simulink model "six_pulse_dstack_based_rectifier"  (R2026a)
settings: Solver=ode23tb  StopTime=simlength  FixedStep=Ts  MaxStep=Tc  EnableMultiTasking=on
values from neighbouring files (symbols this model uses):
  Csnubber = 0.1e-6    (= 1e-07)    [init_model.m]
  LFu_dc = 1.2e-3    (= 0.0012)    [init_model.m]
  Rgrading = 2.4e6    (= 2400000)    [init_model.m]
  RLFu_dc = 2e-4    (= 0.0002)    [init_model.m]
  Rsnubber = 1000    [init_model.m]
  Tc = Tcontrol_rect/4000    (= 5e-08)    [init_model.m]
  Tcontrol_rect = tPWM_RECT    (= 0.0002)    [init_model.m]
  Vnom_ac_adc = 400/sqrt(3)*sqrt(2)    [init_model.m]
  w_grid = f_grid*2*pi    (= 314.159265359)    [init_model.m]
undefined symbols (not defined in the file or in its folder): magnitude, rms
libraries: fl_lib x179, nesl_utility x129, diode_rr_lib x36, ee_lib x2
(part 2 of 5)

== system six_pulse_dstack_based_rectifier/six_pulse rectifier/BR2/ssc_diode_rr_bridge/D1/D12 ==
  D12 : Subsystem
      settings: PortSchema="{\"entries\":[{\"content\":{\"sides\":[{\"content\":{},\"type\":\"ConnectorPlacement.EquallySpacedRectSide\",\"uuid\":\"7269b907-ab9b-4481-ac18-a8dd984c3818\"},{\"content\":{\"side\":\"RIGHT\"},\"type\":\"ConnectorPlacement.EquallySpacedRectSide\",\"uuid\":\"8dceca02-62a3-4342-b624-c7d4418298d0\"},{\"content\":{\"connectorIds\":[\"LConn1\"],\"side\":\"TOP\"},\"type\":\"ConnectorPlacement.EquallySpacedRectSide\",\"uuid\":\"a3401fa4-31f5-4c91-8a09-9f2730c54d6f\"},{\"content\":{\"connectorIds\":[\"RConn1\"],\"side\":\"BOTTOM\"},\"type\":\"ConnectorPlacement.EquallySpacedRectSide\",\"uuid\":\"ec3e6ca2-4822-4b63-8ee1-1049d14efe1d\"}]},\"type\":\"ConnectorPlacement.EquallySpacedConnector\",\"uuid\":\"06f44f8b-bef4-44e1-af36-23832e4d595a\"}],\"packageUris\":[\"http://schema.mathworks.com/mf0/Connector/R2020b\"],\"version\":\"1.0\"}"
  K : PMIOPort  Side=Right
  A : PMIOPort  Port=2  Side=Left
  connections:
  A/RConn1 -- D12/RConn1
  D12/LConn1 -- K/RConn1

== system six_pulse_dstack_based_rectifier/six_pulse rectifier/BR2/ssc_diode_rr_bridge/D1/D13 ==
  D13 : Subsystem
      settings: PortSchema="{\"entries\":[{\"content\":{\"sides\":[{\"content\":{},\"type\":\"ConnectorPlacement.EquallySpacedRectSide\",\"uuid\":\"7269b907-ab9b-4481-ac18-a8dd984c3818\"},{\"content\":{\"side\":\"RIGHT\"},\"type\":\"ConnectorPlacement.EquallySpacedRectSide\",\"uuid\":\"8dceca02-62a3-4342-b624-c7d4418298d0\"},{\"content\":{\"connectorIds\":[\"LConn1\"],\"side\":\"TOP\"},\"type\":\"ConnectorPlacement.EquallySpacedRectSide\",\"uuid\":\"a3401fa4-31f5-4c91-8a09-9f2730c54d6f\"},{\"content\":{\"connectorIds\":[\"RConn1\"],\"side\":\"BOTTOM\"},\"type\":\"ConnectorPlacement.EquallySpacedRectSide\",\"uuid\":\"ec3e6ca2-4822-4b63-8ee1-1049d14efe1d\"}]},\"type\":\"ConnectorPlacement.EquallySpacedConnector\",\"uuid\":\"06f44f8b-bef4-44e1-af36-23832e4d595a\"}],\"packageUris\":[\"http://schema.mathworks.com/mf0/Connector/R2020b\"],\"version\":\"1.0\"}"
  K : PMIOPort  Side=Right
  A : PMIOPort  Port=2  Side=Left
  connections:
  D13/LConn1 -- K/RConn1
  A/RConn1 -- D13/RConn1

== system six_pulse_dstack_based_rectifier/six_pulse rectifier/BR2/ssc_diode_rr_bridge/D1/D14 ==
  D14 : Subsystem
      settings: PortSchema="{\"entries\":[{\"content\":{\"sides\":[{\"content\":{},\"type\":\"ConnectorPlacement.EquallySpacedRectSide\",\"uuid\":\"7269b907-ab9b-4481-ac18-a8dd984c3818\"},{\"content\":{\"side\":\"RIGHT\"},\"type\":\"ConnectorPlacement.EquallySpacedRectSide\",\"uuid\":\"8dceca02-62a3-4342-b624-c7d4418298d0\"},{\"content\":{\"connectorIds\":[\"LConn1\"],\"side\":\"TOP\"},\"type\":\"ConnectorPlacement.EquallySpacedRectSide\",\"uuid\":\"a3401fa4-31f5-4c91-8a09-9f2730c54d6f\"},{\"content\":{\"connectorIds\":[\"RConn1\"],\"side\":\"BOTTOM\"},\"type\":\"ConnectorPlacement.EquallySpacedRectSide\",\"uuid\":\"ec3e6ca2-4822-4b63-8ee1-1049d14efe1d\"}]},\"type\":\"ConnectorPlacement.EquallySpacedConnector\",\"uuid\":\"06f44f8b-bef4-44e1-af36-23832e4d595a\"}],\"packageUris\":[\"http://schema.mathworks.com/mf0/Connector/R2020b\"],\"version\":\"1.0\"}"
  K : PMIOPort  Side=Right
  A : PMIOPort  Port=2  Side=Left
  connections:
  A/RConn1 -- D14/RConn1
  D14/LConn1 -- K/RConn1

== system six_pulse_dstack_based_rectifier/six_pulse rectifier/BR2/ssc_diode_rr_bridge/D1/D15 ==
  D15 : Subsystem
      settings: PortSchema="{\"entries\":[{\"content\":{\"sides\":[{\"content\":{},\"type\":\"ConnectorPlacement.EquallySpacedRectSide\",\"uuid\":\"7269b907-ab9b-4481-ac18-a8dd984c3818\"},{\"content\":{\"side\":\"RIGHT\"},\"type\":\"ConnectorPlacement.EquallySpacedRectSide\",\"uuid\":\"8dceca02-62a3-4342-b624-c7d4418298d0\"},{\"content\":{\"connectorIds\":[\"LConn1\"],\"side\":\"TOP\"},\"type\":\"ConnectorPlacement.EquallySpacedRectSide\",\"uuid\":\"a3401fa4-31f5-4c91-8a09-9f2730c54d6f\"},{\"content\":{\"connectorIds\":[\"RConn1\"],\"side\":\"BOTTOM\"},\"type\":\"ConnectorPlacement.EquallySpacedRectSide\",\"uuid\":\"ec3e6ca2-4822-4b63-8ee1-1049d14efe1d\"}]},\"type\":\"ConnectorPlacement.EquallySpacedConnector\",\"uuid\":\"06f44f8b-bef4-44e1-af36-23832e4d595a\"}],\"packageUris\":[\"http://schema.mathworks.com/mf0/Connector/R2020b\"],\"version\":\"1.0\"}"
  K : PMIOPort  Side=Right
  A : PMIOPort  Port=2  Side=Left
  connections:
  D15/LConn1 -- K/RConn1
  A/RConn1 -- D15/RConn1

== system six_pulse_dstack_based_rectifier/six_pulse rectifier/BR2/ssc_diode_rr_bridge/D1/D16 ==
  D16 : Subsystem
      settings: PortSchema="{\"entries\":[{\"content\":{\"sides\":[{\"content\":{},\"type\":\"ConnectorPlacement.EquallySpacedRectSide\",\"uuid\":\"7269b907-ab9b-4481-ac18-a8dd984c3818\"},{\"content\":{\"side\":\"RIGHT\"},\"type\":\"ConnectorPlacement.EquallySpacedRectSide\",\"uuid\":\"8dceca02-62a3-4342-b624-c7d4418298d0\"},{\"content\":{\"connectorIds\":[\"LConn1\"],\"side\":\"TOP\"},\"type\":\"ConnectorPlacement.EquallySpacedRectSide\",\"uuid\":\"a3401fa4-31f5-4c91-8a09-9f2730c54d6f\"},{\"content\":{\"connectorIds\":[\"RConn1\"],\"side\":\"BOTTOM\"},\"type\":\"ConnectorPlacement.EquallySpacedRectSide\",\"uuid\":\"ec3e6ca2-4822-4b63-8ee1-1049d14efe1d\"}]},\"type\":\"ConnectorPlacement.EquallySpacedConnector\",\"uuid\":\"06f44f8b-bef4-44e1-af36-23832e4d595a\"}],\"packageUris\":[\"http://schema.mathworks.com/mf0/Connector/R2020b\"],\"version\":\"1.0\"}"
  K : PMIOPort  Side=Right
  A : PMIOPort  Port=2  Side=Left
  connections:
  A/RConn1 -- D16/RConn1
  D16/LConn1 -- K/RConn1

== system six_pulse_dstack_based_rectifier/six_pulse rectifier/BR2/ssc_diode_rr_bridge/D1/Rgrading ==
  Current Sensor : fl_lib/Electrical/Electrical Sensors/Current Sensor
  PS-Simulink Converter : nesl_utility/PS-Simulink Converter  PhysicalDomain=network_engine_domain  SubClassName=ps_output  LeftPortType=input  RightPortType=output  PseudoPeriodic=off  Frequencies=[]  VectorFormat=inherit  Unit=inherit  AffineConversion=off
  PS-Simulink Converter1 : nesl_utility/PS-Simulink Converter  PhysicalDomain=network_engine_domain  SubClassName=ps_output  LeftPortType=input  RightPortType=output  PseudoPeriodic=off  Frequencies=[]  VectorFormat=inherit  Unit=inherit  AffineConversion=off
  R11 : fl_lib/Electrical/Electrical Elements/Resistor  R=Rgrading_m Ohm  i_specify=off  i_priority=None  i=0 A  i_nominal_specify=off  i_nominal_value=1  i_nominal_unit=A  v_specify=off  v_priority=None  v=0 V  v_nominal_specify=off  v_nominal_value=1  v_nominal_unit=V
  Voltage Sensor : fl_lib/Electrical/Electrical Sensors/Voltage Sensor
  K : PMIOPort  Side=Right
  A : PMIOPort  Port=2  Side=Left
  tag scope: Rg11_I=scoped, Rg11_U=scoped
  wires:
  PS-Simulink Converter/1 -> [Rg11_U]
  PS-Simulink Converter1/1 -> [Rg11_I]
  connections:
  Voltage Sensor/LConn1 -- Current Sensor/LConn1 -- A/RConn1
  R11/RConn1 -- Voltage Sensor/RConn2 -- K/RConn1
  PS-Simulink Converter/LConn1 -- Voltage Sensor/RConn1
  Current Sensor/RConn2 -- R11/LConn1
  Current Sensor/RConn1 -- PS-Simulink Converter1/LConn1

== system six_pulse_dstack_based_rectifier/six_pulse rectifier/BR2/ssc_diode_rr_bridge/D2/D11 ==
  D11 : Subsystem
      settings: PortSchema="{\"entries\":[{\"content\":{\"sides\":[{\"content\":{},\"type\":\"ConnectorPlacement.EquallySpacedRectSide\",\"uuid\":\"7269b907-ab9b-4481-ac18-a8dd984c3818\"},{\"content\":{\"side\":\"RIGHT\"},\"type\":\"ConnectorPlacement.EquallySpacedRectSide\",\"uuid\":\"8dceca02-62a3-4342-b624-c7d4418298d0\"},{\"content\":{\"connectorIds\":[\"LConn1\"],\"side\":\"TOP\"},\"type\":\"ConnectorPlacement.EquallySpacedRectSide\",\"uuid\":\"a3401fa4-31f5-4c91-8a09-9f2730c54d6f\"},{\"content\":{\"connectorIds\":[\"RConn1\"],\"side\":\"BOTTOM\"},\"type\":\"ConnectorPlacement.EquallySpacedRectSide\",\"uuid\":\"ec3e6ca2-4822-4b63-8ee1-1049d14efe1d\"}]},\"type\":\"ConnectorPlacement.EquallySpacedConnector\",\"uuid\":\"06f44f8b-bef4-44e1-af36-23832e4d595a\"}],\"packageUris\":[\"http://schema.mathworks.com/mf0/Connector/R2020b\"],\"version\":\"1.0\"}"
  K : PMIOPort  Side=Right
  A : PMIOPort  Port=2  Side=Left
  connections:
  A/RConn1 -- D11/RConn1
  D11/LConn1 -- K/RConn1

== system six_pulse_dstack_based_rectifier/six_pulse rectifier/BR2/ssc_diode_rr_bridge/D2/D12 ==
  D12 : Subsystem
      settings: PortSchema="{\"entries\":[{\"content\":{\"sides\":[{\"content\":{},\"type\":\"ConnectorPlacement.EquallySpacedRectSide\",\"uuid\":\"7269b907-ab9b-4481-ac18-a8dd984c3818\"},{\"content\":{\"side\":\"RIGHT\"},\"type\":\"ConnectorPlacement.EquallySpacedRectSide\",\"uuid\":\"8dceca02-62a3-4342-b624-c7d4418298d0\"},{\"content\":{\"connectorIds\":[\"LConn1\"],\"side\":\"TOP\"},\"type\":\"ConnectorPlacement.EquallySpacedRectSide\",\"uuid\":\"a3401fa4-31f5-4c91-8a09-9f2730c54d6f\"},{\"content\":{\"connectorIds\":[\"RConn1\"],\"side\":\"BOTTOM\"},\"type\":\"ConnectorPlacement.EquallySpacedRectSide\",\"uuid\":\"ec3e6ca2-4822-4b63-8ee1-1049d14efe1d\"}]},\"type\":\"ConnectorPlacement.EquallySpacedConnector\",\"uuid\":\"06f44f8b-bef4-44e1-af36-23832e4d595a\"}],\"packageUris\":[\"http://schema.mathworks.com/mf0/Connector/R2020b\"],\"version\":\"1.0\"}"
  K : PMIOPort  Side=Right
  A : PMIOPort  Port=2  Side=Left
  connections:
  D12/LConn1 -- K/RConn1
  A/RConn1 -- D12/RConn1

== system six_pulse_dstack_based_rectifier/six_pulse rectifier/BR2/ssc_diode_rr_bridge/D2/D13 ==
  D13 : Subsystem
      settings: PortSchema="{\"entries\":[{\"content\":{\"sides\":[{\"content\":{},\"type\":\"ConnectorPlacement.EquallySpacedRectSide\",\"uuid\":\"7269b907-ab9b-4481-ac18-a8dd984c3818\"},{\"content\":{\"side\":\"RIGHT\"},\"type\":\"ConnectorPlacement.EquallySpacedRectSide\",\"uuid\":\"8dceca02-62a3-4342-b624-c7d4418298d0\"},{\"content\":{\"connectorIds\":[\"LConn1\"],\"side\":\"TOP\"},\"type\":\"ConnectorPlacement.EquallySpacedRectSide\",\"uuid\":\"a3401fa4-31f5-4c91-8a09-9f2730c54d6f\"},{\"content\":{\"connectorIds\":[\"RConn1\"],\"side\":\"BOTTOM\"},\"type\":\"ConnectorPlacement.EquallySpacedRectSide\",\"uuid\":\"ec3e6ca2-4822-4b63-8ee1-1049d14efe1d\"}]},\"type\":\"ConnectorPlacement.EquallySpacedConnector\",\"uuid\":\"06f44f8b-bef4-44e1-af36-23832e4d595a\"}],\"packageUris\":[\"http://schema.mathworks.com/mf0/Connector/R2020b\"],\"version\":\"1.0\"}"
  K : PMIOPort  Side=Right
  A : PMIOPort  Port=2  Side=Left
  connections:
  A/RConn1 -- D13/RConn1
  D13/LConn1 -- K/RConn1

== system six_pulse_dstack_based_rectifier/six_pulse rectifier/BR2/ssc_diode_rr_bridge/D2/D14 ==
  D14 : Subsystem
      settings: PortSchema="{\"entries\":[{\"content\":{\"sides\":[{\"content\":{},\"type\":\"ConnectorPlacement.EquallySpacedRectSide\",\"uuid\":\"7269b907-ab9b-4481-ac18-a8dd984c3818\"},{\"content\":{\"side\":\"RIGHT\"},\"type\":\"ConnectorPlacement.EquallySpacedRectSide\",\"uuid\":\"8dceca02-62a3-4342-b624-c7d4418298d0\"},{\"content\":{\"connectorIds\":[\"LConn1\"],\"side\":\"TOP\"},\"type\":\"ConnectorPlacement.EquallySpacedRectSide\",\"uuid\":\"a3401fa4-31f5-4c91-8a09-9f2730c54d6f\"},{\"content\":{\"connectorIds\":[\"RConn1\"],\"side\":\"BOTTOM\"},\"type\":\"ConnectorPlacement.EquallySpacedRectSide\",\"uuid\":\"ec3e6ca2-4822-4b63-8ee1-1049d14efe1d\"}]},\"type\":\"ConnectorPlacement.EquallySpacedConnector\",\"uuid\":\"06f44f8b-bef4-44e1-af36-23832e4d595a\"}],\"packageUris\":[\"http://schema.mathworks.com/mf0/Connector/R2020b\"],\"version\":\"1.0\"}"
  K : PMIOPort  Side=Right
  A : PMIOPort  Port=2  Side=Left
  connections:
  D14/LConn1 -- K/RConn1
  A/RConn1 -- D14/RConn1

== system six_pulse_dstack_based_rectifier/six_pulse rectifier/BR2/ssc_diode_rr_bridge/D2/D15 ==
  D15 : Subsystem
      settings: PortSchema="{\"entries\":[{\"content\":{\"sides\":[{\"content\":{},\"type\":\"ConnectorPlacement.EquallySpacedRectSide\",\"uuid\":\"7269b907-ab9b-4481-ac18-a8dd984c3818\"},{\"content\":{\"side\":\"RIGHT\"},\"type\":\"ConnectorPlacement.EquallySpacedRectSide\",\"uuid\":\"8dceca02-62a3-4342-b624-c7d4418298d0\"},{\"content\":{\"connectorIds\":[\"LConn1\"],\"side\":\"TOP\"},\"type\":\"ConnectorPlacement.EquallySpacedRectSide\",\"uuid\":\"a3401fa4-31f5-4c91-8a09-9f2730c54d6f\"},{\"content\":{\"connectorIds\":[\"RConn1\"],\"side\":\"BOTTOM\"},\"type\":\"ConnectorPlacement.EquallySpacedRectSide\",\"uuid\":\"ec3e6ca2-4822-4b63-8ee1-1049d14efe1d\"}]},\"type\":\"ConnectorPlacement.EquallySpacedConnector\",\"uuid\":\"06f44f8b-bef4-44e1-af36-23832e4d595a\"}],\"packageUris\":[\"http://schema.mathworks.com/mf0/Connector/R2020b\"],\"version\":\"1.0\"}"
  K : PMIOPort  Side=Right
  A : PMIOPort  Port=2  Side=Left
  connections:
  A/RConn1 -- D15/RConn1
  D15/LConn1 -- K/RConn1

== system six_pulse_dstack_based_rectifier/six_pulse rectifier/BR2/ssc_diode_rr_bridge/D2/D16 ==
  D16 : Subsystem
      settings: PortSchema="{\"entries\":[{\"content\":{\"sides\":[{\"content\":{},\"type\":\"ConnectorPlacement.EquallySpacedRectSide\",\"uuid\":\"7269b907-ab9b-4481-ac18-a8dd984c3818\"},{\"content\":{\"side\":\"RIGHT\"},\"type\":\"ConnectorPlacement.EquallySpacedRectSide\",\"uuid\":\"8dceca02-62a3-4342-b624-c7d4418298d0\"},{\"content\":{\"connectorIds\":[\"LConn1\"],\"side\":\"TOP\"},\"type\":\"ConnectorPlacement.EquallySpacedRectSide\",\"uuid\":\"a3401fa4-31f5-4c91-8a09-9f2730c54d6f\"},{\"content\":{\"connectorIds\":[\"RConn1\"],\"side\":\"BOTTOM\"},\"type\":\"ConnectorPlacement.EquallySpacedRectSide\",\"uuid\":\"ec3e6ca2-4822-4b63-8ee1-1049d14efe1d\"}]},\"type\":\"ConnectorPlacement.EquallySpacedConnector\",\"uuid\":\"06f44f8b-bef4-44e1-af36-23832e4d595a\"}],\"packageUris\":[\"http://schema.mathworks.com/mf0/Connector/R2020b\"],\"version\":\"1.0\"}"
  K : PMIOPort  Side=Right
  A : PMIOPort  Port=2  Side=Left
  connections:
  D16/LConn1 -- K/RConn1
  A/RConn1 -- D16/RConn1

== system six_pulse_dstack_based_rectifier/six_pulse rectifier/BR2/ssc_diode_rr_bridge/D3/D11 ==
  D11 : Subsystem
      settings: PortSchema="{\"entries\":[{\"content\":{\"sides\":[{\"content\":{},\"type\":\"ConnectorPlacement.EquallySpacedRectSide\",\"uuid\":\"7269b907-ab9b-4481-ac18-a8dd984c3818\"},{\"content\":{\"side\":\"RIGHT\"},\"type\":\"ConnectorPlacement.EquallySpacedRectSide\",\"uuid\":\"8dceca02-62a3-4342-b624-c7d4418298d0\"},{\"content\":{\"connectorIds\":[\"LConn1\"],\"side\":\"TOP\"},\"type\":\"ConnectorPlacement.EquallySpacedRectSide\",\"uuid\":\"a3401fa4-31f5-4c91-8a09-9f2730c54d6f\"},{\"content\":{\"connectorIds\":[\"RConn1\"],\"side\":\"BOTTOM\"},\"type\":\"ConnectorPlacement.EquallySpacedRectSide\",\"uuid\":\"ec3e6ca2-4822-4b63-8ee1-1049d14efe1d\"}]},\"type\":\"ConnectorPlacement.EquallySpacedConnector\",\"uuid\":\"06f44f8b-bef4-44e1-af36-23832e4d595a\"}],\"packageUris\":[\"http://schema.mathworks.com/mf0/Connector/R2020b\"],\"version\":\"1.0\"}"
  K : PMIOPort  Side=Right
  A : PMIOPort  Port=2  Side=Left
  connections:
  A/RConn1 -- D11/RConn1
  D11/LConn1 -- K/RConn1

== system six_pulse_dstack_based_rectifier/six_pulse rectifier/BR2/ssc_diode_rr_bridge/D3/D12 ==
  D12 : Subsystem
      settings: PortSchema="{\"entries\":[{\"content\":{\"sides\":[{\"content\":{},\"type\":\"ConnectorPlacement.EquallySpacedRectSide\",\"uuid\":\"7269b907-ab9b-4481-ac18-a8dd984c3818\"},{\"content\":{\"side\":\"RIGHT\"},\"type\":\"ConnectorPlacement.EquallySpacedRectSide\",\"uuid\":\"8dceca02-62a3-4342-b624-c7d4418298d0\"},{\"content\":{\"connectorIds\":[\"LConn1\"],\"side\":\"TOP\"},\"type\":\"ConnectorPlacement.EquallySpacedRectSide\",\"uuid\":\"a3401fa4-31f5-4c91-8a09-9f2730c54d6f\"},{\"content\":{\"connectorIds\":[\"RConn1\"],\"side\":\"BOTTOM\"},\"type\":\"ConnectorPlacement.EquallySpacedRectSide\",\"uuid\":\"ec3e6ca2-4822-4b63-8ee1-1049d14efe1d\"}]},\"type\":\"ConnectorPlacement.EquallySpacedConnector\",\"uuid\":\"06f44f8b-bef4-44e1-af36-23832e4d595a\"}],\"packageUris\":[\"http://schema.mathworks.com/mf0/Connector/R2020b\"],\"version\":\"1.0\"}"
  K : PMIOPort  Side=Right
  A : PMIOPort  Port=2  Side=Left
  connections:
  D12/LConn1 -- K/RConn1
  A/RConn1 -- D12/RConn1

== system six_pulse_dstack_based_rectifier/six_pulse rectifier/BR2/ssc_diode_rr_bridge/D3/D13 ==
  D13 : Subsystem
      settings: PortSchema="{\"entries\":[{\"content\":{\"sides\":[{\"content\":{},\"type\":\"ConnectorPlacement.EquallySpacedRectSide\",\"uuid\":\"7269b907-ab9b-4481-ac18-a8dd984c3818\"},{\"content\":{\"side\":\"RIGHT\"},\"type\":\"ConnectorPlacement.EquallySpacedRectSide\",\"uuid\":\"8dceca02-62a3-4342-b624-c7d4418298d0\"},{\"content\":{\"connectorIds\":[\"LConn1\"],\"side\":\"TOP\"},\"type\":\"ConnectorPlacement.EquallySpacedRectSide\",\"uuid\":\"a3401fa4-31f5-4c91-8a09-9f2730c54d6f\"},{\"content\":{\"connectorIds\":[\"RConn1\"],\"side\":\"BOTTOM\"},\"type\":\"ConnectorPlacement.EquallySpacedRectSide\",\"uuid\":\"ec3e6ca2-4822-4b63-8ee1-1049d14efe1d\"}]},\"type\":\"ConnectorPlacement.EquallySpacedConnector\",\"uuid\":\"06f44f8b-bef4-44e1-af36-23832e4d595a\"}],\"packageUris\":[\"http://schema.mathworks.com/mf0/Connector/R2020b\"],\"version\":\"1.0\"}"
  K : PMIOPort  Side=Right
  A : PMIOPort  Port=2  Side=Left
  connections:
  A/RConn1 -- D13/RConn1
  D13/LConn1 -- K/RConn1

== system six_pulse_dstack_based_rectifier/six_pulse rectifier/BR2/ssc_diode_rr_bridge/D3/D14 ==
  D14 : Subsystem
      settings: PortSchema="{\"entries\":[{\"content\":{\"sides\":[{\"content\":{},\"type\":\"ConnectorPlacement.EquallySpacedRectSide\",\"uuid\":\"7269b907-ab9b-4481-ac18-a8dd984c3818\"},{\"content\":{\"side\":\"RIGHT\"},\"type\":\"ConnectorPlacement.EquallySpacedRectSide\",\"uuid\":\"8dceca02-62a3-4342-b624-c7d4418298d0\"},{\"content\":{\"connectorIds\":[\"LConn1\"],\"side\":\"TOP\"},\"type\":\"ConnectorPlacement.EquallySpacedRectSide\",\"uuid\":\"a3401fa4-31f5-4c91-8a09-9f2730c54d6f\"},{\"content\":{\"connectorIds\":[\"RConn1\"],\"side\":\"BOTTOM\"},\"type\":\"ConnectorPlacement.EquallySpacedRectSide\",\"uuid\":\"ec3e6ca2-4822-4b63-8ee1-1049d14efe1d\"}]},\"type\":\"ConnectorPlacement.EquallySpacedConnector\",\"uuid\":\"06f44f8b-bef4-44e1-af36-23832e4d595a\"}],\"packageUris\":[\"http://schema.mathworks.com/mf0/Connector/R2020b\"],\"version\":\"1.0\"}"
  K : PMIOPort  Side=Right
  A : PMIOPort  Port=2  Side=Left
  connections:
  D14/LConn1 -- K/RConn1
  A/RConn1 -- D14/RConn1

== system six_pulse_dstack_based_rectifier/six_pulse rectifier/BR2/ssc_diode_rr_bridge/D3/D15 ==
  D15 : Subsystem
      settings: PortSchema="{\"entries\":[{\"content\":{\"sides\":[{\"content\":{},\"type\":\"ConnectorPlacement.EquallySpacedRectSide\",\"uuid\":\"7269b907-ab9b-4481-ac18-a8dd984c3818\"},{\"content\":{\"side\":\"RIGHT\"},\"type\":\"ConnectorPlacement.EquallySpacedRectSide\",\"uuid\":\"8dceca02-62a3-4342-b624-c7d4418298d0\"},{\"content\":{\"connectorIds\":[\"LConn1\"],\"side\":\"TOP\"},\"type\":\"ConnectorPlacement.EquallySpacedRectSide\",\"uuid\":\"a3401fa4-31f5-4c91-8a09-9f2730c54d6f\"},{\"content\":{\"connectorIds\":[\"RConn1\"],\"side\":\"BOTTOM\"},\"type\":\"ConnectorPlacement.EquallySpacedRectSide\",\"uuid\":\"ec3e6ca2-4822-4b63-8ee1-1049d14efe1d\"}]},\"type\":\"ConnectorPlacement.EquallySpacedConnector\",\"uuid\":\"06f44f8b-bef4-44e1-af36-23832e4d595a\"}],\"packageUris\":[\"http://schema.mathworks.com/mf0/Connector/R2020b\"],\"version\":\"1.0\"}"
  K : PMIOPort  Side=Right
  A : PMIOPort  Port=2  Side=Left
  connections:
  A/RConn1 -- D15/RConn1
  D15/LConn1 -- K/RConn1

== system six_pulse_dstack_based_rectifier/six_pulse rectifier/BR2/ssc_diode_rr_bridge/D3/D16 ==
  D16 : Subsystem
      settings: PortSchema="{\"entries\":[{\"content\":{\"sides\":[{\"content\":{},\"type\":\"ConnectorPlacement.EquallySpacedRectSide\",\"uuid\":\"7269b907-ab9b-4481-ac18-a8dd984c3818\"},{\"content\":{\"side\":\"RIGHT\"},\"type\":\"ConnectorPlacement.EquallySpacedRectSide\",\"uuid\":\"8dceca02-62a3-4342-b624-c7d4418298d0\"},{\"content\":{\"connectorIds\":[\"LConn1\"],\"side\":\"TOP\"},\"type\":\"ConnectorPlacement.EquallySpacedRectSide\",\"uuid\":\"a3401fa4-31f5-4c91-8a09-9f2730c54d6f\"},{\"content\":{\"connectorIds\":[\"RConn1\"],\"side\":\"BOTTOM\"},\"type\":\"ConnectorPlacement.EquallySpacedRectSide\",\"uuid\":\"ec3e6ca2-4822-4b63-8ee1-1049d14efe1d\"}]},\"type\":\"ConnectorPlacement.EquallySpacedConnector\",\"uuid\":\"06f44f8b-bef4-44e1-af36-23832e4d595a\"}],\"packageUris\":[\"http://schema.mathworks.com/mf0/Connector/R2020b\"],\"version\":\"1.0\"}"
  K : PMIOPort  Side=Right
  A : PMIOPort  Port=2  Side=Left
  connections:
  D16/LConn1 -- K/RConn1
  A/RConn1 -- D16/RConn1

== system six_pulse_dstack_based_rectifier/six_pulse rectifier/BR2/ssc_diode_rr_bridge/D4/D11 ==
  D11 : Subsystem
      settings: PortSchema="{\"entries\":[{\"content\":{\"sides\":[{\"content\":{},\"type\":\"ConnectorPlacement.EquallySpacedRectSide\",\"uuid\":\"7269b907-ab9b-4481-ac18-a8dd984c3818\"},{\"content\":{\"side\":\"RIGHT\"},\"type\":\"ConnectorPlacement.EquallySpacedRectSide\",\"uuid\":\"8dceca02-62a3-4342-b624-c7d4418298d0\"},{\"content\":{\"connectorIds\":[\"LConn1\"],\"side\":\"TOP\"},\"type\":\"ConnectorPlacement.EquallySpacedRectSide\",\"uuid\":\"a3401fa4-31f5-4c91-8a09-9f2730c54d6f\"},{\"content\":{\"connectorIds\":[\"RConn1\"],\"side\":\"BOTTOM\"},\"type\":\"ConnectorPlacement.EquallySpacedRectSide\",\"uuid\":\"ec3e6ca2-4822-4b63-8ee1-1049d14efe1d\"}]},\"type\":\"ConnectorPlacement.EquallySpacedConnector\",\"uuid\":\"06f44f8b-bef4-44e1-af36-23832e4d595a\"}],\"packageUris\":[\"http://schema.mathworks.com/mf0/Connector/R2020b\"],\"version\":\"1.0\"}"
  K : PMIOPort  Side=Right
  A : PMIOPort  Port=2  Side=Left
  connections:
  D11/LConn1 -- K/RConn1
  A/RConn1 -- D11/RConn1

== system six_pulse_dstack_based_rectifier/six_pulse rectifier/BR2/ssc_diode_rr_bridge/D4/D12 ==
  D12 : Subsystem
      settings: PortSchema="{\"entries\":[{\"content\":{\"sides\":[{\"content\":{},\"type\":\"ConnectorPlacement.EquallySpacedRectSide\",\"uuid\":\"7269b907-ab9b-4481-ac18-a8dd984c3818\"},{\"content\":{\"side\":\"RIGHT\"},\"type\":\"ConnectorPlacement.EquallySpacedRectSide\",\"uuid\":\"8dceca02-62a3-4342-b624-c7d4418298d0\"},{\"content\":{\"connectorIds\":[\"LConn1\"],\"side\":\"TOP\"},\"type\":\"ConnectorPlacement.EquallySpacedRectSide\",\"uuid\":\"a3401fa4-31f5-4c91-8a09-9f2730c54d6f\"},{\"content\":{\"connectorIds\":[\"RConn1\"],\"side\":\"BOTTOM\"},\"type\":\"ConnectorPlacement.EquallySpacedRectSide\",\"uuid\":\"ec3e6ca2-4822-4b63-8ee1-1049d14efe1d\"}]},\"type\":\"ConnectorPlacement.EquallySpacedConnector\",\"uuid\":\"06f44f8b-bef4-44e1-af36-23832e4d595a\"}],\"packageUris\":[\"http://schema.mathworks.com/mf0/Connector/R2020b\"],\"version\":\"1.0\"}"
  K : PMIOPort  Side=Right
  A : PMIOPort  Port=2  Side=Left
  connections:
  A/RConn1 -- D12/RConn1
  D12/LConn1 -- K/RConn1

== system six_pulse_dstack_based_rectifier/six_pulse rectifier/BR2/ssc_diode_rr_bridge/D4/D13 ==
  D13 : Subsystem
      settings: PortSchema="{\"entries\":[{\"content\":{\"sides\":[{\"content\":{},\"type\":\"ConnectorPlacement.EquallySpacedRectSide\",\"uuid\":\"7269b907-ab9b-4481-ac18-a8dd984c3818\"},{\"content\":{\"side\":\"RIGHT\"},\"type\":\"ConnectorPlacement.EquallySpacedRectSide\",\"uuid\":\"8dceca02-62a3-4342-b624-c7d4418298d0\"},{\"content\":{\"connectorIds\":[\"LConn1\"],\"side\":\"TOP\"},\"type\":\"ConnectorPlacement.EquallySpacedRectSide\",\"uuid\":\"a3401fa4-31f5-4c91-8a09-9f2730c54d6f\"},{\"content\":{\"connectorIds\":[\"RConn1\"],\"side\":\"BOTTOM\"},\"type\":\"ConnectorPlacement.EquallySpacedRectSide\",\"uuid\":\"ec3e6ca2-4822-4b63-8ee1-1049d14efe1d\"}]},\"type\":\"ConnectorPlacement.EquallySpacedConnector\",\"uuid\":\"06f44f8b-bef4-44e1-af36-23832e4d595a\"}],\"packageUris\":[\"http://schema.mathworks.com/mf0/Connector/R2020b\"],\"version\":\"1.0\"}"
  K : PMIOPort  Side=Right
  A : PMIOPort  Port=2  Side=Left
  connections:
  D13/LConn1 -- K/RConn1
  A/RConn1 -- D13/RConn1

== system six_pulse_dstack_based_rectifier/six_pulse rectifier/BR2/ssc_diode_rr_bridge/D4/D14 ==
  D14 : Subsystem
      settings: PortSchema="{\"entries\":[{\"content\":{\"sides\":[{\"content\":{},\"type\":\"ConnectorPlacement.EquallySpacedRectSide\",\"uuid\":\"7269b907-ab9b-4481-ac18-a8dd984c3818\"},{\"content\":{\"side\":\"RIGHT\"},\"type\":\"ConnectorPlacement.EquallySpacedRectSide\",\"uuid\":\"8dceca02-62a3-4342-b624-c7d4418298d0\"},{\"content\":{\"connectorIds\":[\"LConn1\"],\"side\":\"TOP\"},\"type\":\"ConnectorPlacement.EquallySpacedRectSide\",\"uuid\":\"a3401fa4-31f5-4c91-8a09-9f2730c54d6f\"},{\"content\":{\"connectorIds\":[\"RConn1\"],\"side\":\"BOTTOM\"},\"type\":\"ConnectorPlacement.EquallySpacedRectSide\",\"uuid\":\"ec3e6ca2-4822-4b63-8ee1-1049d14efe1d\"}]},\"type\":\"ConnectorPlacement.EquallySpacedConnector\",\"uuid\":\"06f44f8b-bef4-44e1-af36-23832e4d595a\"}],\"packageUris\":[\"http://schema.mathworks.com/mf0/Connector/R2020b\"],\"version\":\"1.0\"}"
  K : PMIOPort  Side=Right
  A : PMIOPort  Port=2  Side=Left
  connections:
  A/RConn1 -- D14/RConn1
  D14/LConn1 -- K/RConn1

== system six_pulse_dstack_based_rectifier/six_pulse rectifier/BR2/ssc_diode_rr_bridge/D4/D15 ==
  D15 : Subsystem
      settings: PortSchema="{\"entries\":[{\"content\":{\"sides\":[{\"content\":{},\"type\":\"ConnectorPlacement.EquallySpacedRectSide\",\"uuid\":\"7269b907-ab9b-4481-ac18-a8dd984c3818\"},{\"content\":{\"side\":\"RIGHT\"},\"type\":\"ConnectorPlacement.EquallySpacedRectSide\",\"uuid\":\"8dceca02-62a3-4342-b624-c7d4418298d0\"},{\"content\":{\"connectorIds\":[\"LConn1\"],\"side\":\"TOP\"},\"type\":\"ConnectorPlacement.EquallySpacedRectSide\",\"uuid\":\"a3401fa4-31f5-4c91-8a09-9f2730c54d6f\"},{\"content\":{\"connectorIds\":[\"RConn1\"],\"side\":\"BOTTOM\"},\"type\":\"ConnectorPlacement.EquallySpacedRectSide\",\"uuid\":\"ec3e6ca2-4822-4b63-8ee1-1049d14efe1d\"}]},\"type\":\"ConnectorPlacement.EquallySpacedConnector\",\"uuid\":\"06f44f8b-bef4-44e1-af36-23832e4d595a\"}],\"packageUris\":[\"http://schema.mathworks.com/mf0/Connector/R2020b\"],\"version\":\"1.0\"}"
  K : PMIOPort  Side=Right
  A : PMIOPort  Port=2  Side=Left
  connections:
  D15/LConn1 -- K/RConn1
  A/RConn1 -- D15/RConn1

== system six_pulse_dstack_based_rectifier/six_pulse rectifier/BR2/ssc_diode_rr_bridge/D4/D16 ==
  D16 : Subsystem
      settings: PortSchema="{\"entries\":[{\"content\":{\"sides\":[{\"content\":{},\"type\":\"ConnectorPlacement.EquallySpacedRectSide\",\"uuid\":\"7269b907-ab9b-4481-ac18-a8dd984c3818\"},{\"content\":{\"side\":\"RIGHT\"},\"type\":\"ConnectorPlacement.EquallySpacedRectSide\",\"uuid\":\"8dceca02-62a3-4342-b624-c7d4418298d0\"},{\"content\":{\"connectorIds\":[\"LConn1\"],\"side\":\"TOP\"},\"type\":\"ConnectorPlacement.EquallySpacedRectSide\",\"uuid\":\"a3401fa4-31f5-4c91-8a09-9f2730c54d6f\"},{\"content\":{\"connectorIds\":[\"RConn1\"],\"side\":\"BOTTOM\"},\"type\":\"ConnectorPlacement.EquallySpacedRectSide\",\"uuid\":\"ec3e6ca2-4822-4b63-8ee1-1049d14efe1d\"}]},\"type\":\"ConnectorPlacement.EquallySpacedConnector\",\"uuid\":\"06f44f8b-bef4-44e1-af36-23832e4d595a\"}],\"packageUris\":[\"http://schema.mathworks.com/mf0/Connector/R2020b\"],\"version\":\"1.0\"}"
  K : PMIOPort  Side=Right
  A : PMIOPort  Port=2  Side=Left
  connections:
  A/RConn1 -- D16/RConn1
  D16/LConn1 -- K/RConn1

== system six_pulse_dstack_based_rectifier/six_pulse rectifier/BR2/ssc_diode_rr_bridge/D5/D11 ==
  D11 : Subsystem
      settings: PortSchema="{\"entries\":[{\"content\":{\"sides\":[{\"content\":{},\"type\":\"ConnectorPlacement.EquallySpacedRectSide\",\"uuid\":\"7269b907-ab9b-4481-ac18-a8dd984c3818\"},{\"content\":{\"side\":\"RIGHT\"},\"type\":\"ConnectorPlacement.EquallySpacedRectSide\",\"uuid\":\"8dceca02-62a3-4342-b624-c7d4418298d0\"},{\"content\":{\"connectorIds\":[\"LConn1\"],\"side\":\"TOP\"},\"type\":\"ConnectorPlacement.EquallySpacedRectSide\",\"uuid\":\"a3401fa4-31f5-4c91-8a09-9f2730c54d6f\"},{\"content\":{\"connectorIds\":[\"RConn1\"],\"side\":\"BOTTOM\"},\"type\":\"ConnectorPlacement.EquallySpacedRectSide\",\"uuid\":\"ec3e6ca2-4822-4b63-8ee1-1049d14efe1d\"}]},\"type\":\"ConnectorPlacement.EquallySpacedConnector\",\"uuid\":\"06f44f8b-bef4-44e1-af36-23832e4d595a\"}],\"packageUris\":[\"http://schema.mathworks.com/mf0/Connector/R2020b\"],\"version\":\"1.0\"}"
  K : PMIOPort  Side=Right
  A : PMIOPort  Port=2  Side=Left
  connections:
  D11/LConn1 -- K/RConn1
  A/RConn1 -- D11/RConn1

== system six_pulse_dstack_based_rectifier/six_pulse rectifier/BR2/ssc_diode_rr_bridge/D5/D12 ==
  D12 : Subsystem
      settings: PortSchema="{\"entries\":[{\"content\":{\"sides\":[{\"content\":{},\"type\":\"ConnectorPlacement.EquallySpacedRectSide\",\"uuid\":\"7269b907-ab9b-4481-ac18-a8dd984c3818\"},{\"content\":{\"side\":\"RIGHT\"},\"type\":\"ConnectorPlacement.EquallySpacedRectSide\",\"uuid\":\"8dceca02-62a3-4342-b624-c7d4418298d0\"},{\"content\":{\"connectorIds\":[\"LConn1\"],\"side\":\"TOP\"},\"type\":\"ConnectorPlacement.EquallySpacedRectSide\",\"uuid\":\"a3401fa4-31f5-4c91-8a09-9f2730c54d6f\"},{\"content\":{\"connectorIds\":[\"RConn1\"],\"side\":\"BOTTOM\"},\"type\":\"ConnectorPlacement.EquallySpacedRectSide\",\"uuid\":\"ec3e6ca2-4822-4b63-8ee1-1049d14efe1d\"}]},\"type\":\"ConnectorPlacement.EquallySpacedConnector\",\"uuid\":\"06f44f8b-bef4-44e1-af36-23832e4d595a\"}],\"packageUris\":[\"http://schema.mathworks.com/mf0/Connector/R2020b\"],\"version\":\"1.0\"}"
  K : PMIOPort  Side=Right
  A : PMIOPort  Port=2  Side=Left
  connections:
  A/RConn1 -- D12/RConn1
  D12/LConn1 -- K/RConn1

== system six_pulse_dstack_based_rectifier/six_pulse rectifier/BR2/ssc_diode_rr_bridge/D5/D13 ==
  D13 : Subsystem
      settings: PortSchema="{\"entries\":[{\"content\":{\"sides\":[{\"content\":{},\"type\":\"ConnectorPlacement.EquallySpacedRectSide\",\"uuid\":\"7269b907-ab9b-4481-ac18-a8dd984c3818\"},{\"content\":{\"side\":\"RIGHT\"},\"type\":\"ConnectorPlacement.EquallySpacedRectSide\",\"uuid\":\"8dceca02-62a3-4342-b624-c7d4418298d0\"},{\"content\":{\"connectorIds\":[\"LConn1\"],\"side\":\"TOP\"},\"type\":\"ConnectorPlacement.EquallySpacedRectSide\",\"uuid\":\"a3401fa4-31f5-4c91-8a09-9f2730c54d6f\"},{\"content\":{\"connectorIds\":[\"RConn1\"],\"side\":\"BOTTOM\"},\"type\":\"ConnectorPlacement.EquallySpacedRectSide\",\"uuid\":\"ec3e6ca2-4822-4b63-8ee1-1049d14efe1d\"}]},\"type\":\"ConnectorPlacement.EquallySpacedConnector\",\"uuid\":\"06f44f8b-bef4-44e1-af36-23832e4d595a\"}],\"packageUris\":[\"http://schema.mathworks.com/mf0/Connector/R2020b\"],\"version\":\"1.0\"}"
  K : PMIOPort  Side=Right
  A : PMIOPort  Port=2  Side=Left
  connections:
  D13/LConn1 -- K/RConn1
  A/RConn1 -- D13/RConn1

== system six_pulse_dstack_based_rectifier/six_pulse rectifier/BR2/ssc_diode_rr_bridge/D5/D14 ==
  D14 : Subsystem
      settings: PortSchema="{\"entries\":[{\"content\":{\"sides\":[{\"content\":{},\"type\":\"ConnectorPlacement.EquallySpacedRectSide\",\"uuid\":\"7269b907-ab9b-4481-ac18-a8dd984c3818\"},{\"content\":{\"side\":\"RIGHT\"},\"type\":\"ConnectorPlacement.EquallySpacedRectSide\",\"uuid\":\"8dceca02-62a3-4342-b624-c7d4418298d0\"},{\"content\":{\"connectorIds\":[\"LConn1\"],\"side\":\"TOP\"},\"type\":\"ConnectorPlacement.EquallySpacedRectSide\",\"uuid\":\"a3401fa4-31f5-4c91-8a09-9f2730c54d6f\"},{\"content\":{\"connectorIds\":[\"RConn1\"],\"side\":\"BOTTOM\"},\"type\":\"ConnectorPlacement.EquallySpacedRectSide\",\"uuid\":\"ec3e6ca2-4822-4b63-8ee1-1049d14efe1d\"}]},\"type\":\"ConnectorPlacement.EquallySpacedConnector\",\"uuid\":\"06f44f8b-bef4-44e1-af36-23832e4d595a\"}],\"packageUris\":[\"http://schema.mathworks.com/mf0/Connector/R2020b\"],\"version\":\"1.0\"}"
  K : PMIOPort  Side=Right
  A : PMIOPort  Port=2  Side=Left
  connections:
  A/RConn1 -- D14/RConn1
  D14/LConn1 -- K/RConn1

== system six_pulse_dstack_based_rectifier/six_pulse rectifier/BR2/ssc_diode_rr_bridge/D5/D15 ==
  D15 : Subsystem
      settings: PortSchema="{\"entries\":[{\"content\":{\"sides\":[{\"content\":{},\"type\":\"ConnectorPlacement.EquallySpacedRectSide\",\"uuid\":\"7269b907-ab9b-4481-ac18-a8dd984c3818\"},{\"content\":{\"side\":\"RIGHT\"},\"type\":\"ConnectorPlacement.EquallySpacedRectSide\",\"uuid\":\"8dceca02-62a3-4342-b624-c7d4418298d0\"},{\"content\":{\"connectorIds\":[\"LConn1\"],\"side\":\"TOP\"},\"type\":\"ConnectorPlacement.EquallySpacedRectSide\",\"uuid\":\"a3401fa4-31f5-4c91-8a09-9f2730c54d6f\"},{\"content\":{\"connectorIds\":[\"RConn1\"],\"side\":\"BOTTOM\"},\"type\":\"ConnectorPlacement.EquallySpacedRectSide\",\"uuid\":\"ec3e6ca2-4822-4b63-8ee1-1049d14efe1d\"}]},\"type\":\"ConnectorPlacement.EquallySpacedConnector\",\"uuid\":\"06f44f8b-bef4-44e1-af36-23832e4d595a\"}],\"packageUris\":[\"http://schema.mathworks.com/mf0/Connector/R2020b\"],\"version\":\"1.0\"}"
  K : PMIOPort  Side=Right
  A : PMIOPort  Port=2  Side=Left
  connections:
  D15/LConn1 -- K/RConn1
  A/RConn1 -- D15/RConn1

== system six_pulse_dstack_based_rectifier/six_pulse rectifier/BR2/ssc_diode_rr_bridge/D5/D16 ==
  D16 : Subsystem
      settings: PortSchema="{\"entries\":[{\"content\":{\"sides\":[{\"content\":{},\"type\":\"ConnectorPlacement.EquallySpacedRectSide\",\"uuid\":\"7269b907-ab9b-4481-ac18-a8dd984c3818\"},{\"content\":{\"side\":\"RIGHT\"},\"type\":\"ConnectorPlacement.EquallySpacedRectSide\",\"uuid\":\"8dceca02-62a3-4342-b624-c7d4418298d0\"},{\"content\":{\"connectorIds\":[\"LConn1\"],\"side\":\"TOP\"},\"type\":\"ConnectorPlacement.EquallySpacedRectSide\",\"uuid\":\"a3401fa4-31f5-4c91-8a09-9f2730c54d6f\"},{\"content\":{\"connectorIds\":[\"RConn1\"],\"side\":\"BOTTOM\"},\"type\":\"ConnectorPlacement.EquallySpacedRectSide\",\"uuid\":\"ec3e6ca2-4822-4b63-8ee1-1049d14efe1d\"}]},\"type\":\"ConnectorPlacement.EquallySpacedConnector\",\"uuid\":\"06f44f8b-bef4-44e1-af36-23832e4d595a\"}],\"packageUris\":[\"http://schema.mathworks.com/mf0/Connector/R2020b\"],\"version\":\"1.0\"}"
  K : PMIOPort  Side=Right
  A : PMIOPort  Port=2  Side=Left
  connections:
  A/RConn1 -- D16/RConn1
  D16/LConn1 -- K/RConn1

== system six_pulse_dstack_based_rectifier/six_pulse rectifier/BR2/ssc_diode_rr_bridge/D6/D11 ==
  D11 : Subsystem
      settings: PortSchema="{\"entries\":[{\"content\":{\"sides\":[{\"content\":{},\"type\":\"ConnectorPlacement.EquallySpacedRectSide\",\"uuid\":\"7269b907-ab9b-4481-ac18-a8dd984c3818\"},{\"content\":{\"side\":\"RIGHT\"},\"type\":\"ConnectorPlacement.EquallySpacedRectSide\",\"uuid\":\"8dceca02-62a3-4342-b624-c7d4418298d0\"},{\"content\":{\"connectorIds\":[\"LConn1\"],\"side\":\"TOP\"},\"type\":\"ConnectorPlacement.EquallySpacedRectSide\",\"uuid\":\"a3401fa4-31f5-4c91-8a09-9f2730c54d6f\"},{\"content\":{\"connectorIds\":[\"RConn1\"],\"side\":\"BOTTOM\"},\"type\":\"ConnectorPlacement.EquallySpacedRectSide\",\"uuid\":\"ec3e6ca2-4822-4b63-8ee1-1049d14efe1d\"}]},\"type\":\"ConnectorPlacement.EquallySpacedConnector\",\"uuid\":\"06f44f8b-bef4-44e1-af36-23832e4d595a\"}],\"packageUris\":[\"http://schema.mathworks.com/mf0/Connector/R2020b\"],\"version\":\"1.0\"}"
  K : PMIOPort  Side=Right
  A : PMIOPort  Port=2  Side=Left
  connections:
  A/RConn1 -- D11/RConn1
  D11/LConn1 -- K/RConn1

== system six_pulse_dstack_based_rectifier/six_pulse rectifier/BR2/ssc_diode_rr_bridge/D6/D12 ==
  D12 : Subsystem
      settings: PortSchema="{\"entries\":[{\"content\":{\"sides\":[{\"content\":{},\"type\":\"ConnectorPlacement.EquallySpacedRectSide\",\"uuid\":\"7269b907-ab9b-4481-ac18-a8dd984c3818\"},{\"content\":{\"side\":\"RIGHT\"},\"type\":\"ConnectorPlacement.EquallySpacedRectSide\",\"uuid\":\"8dceca02-62a3-4342-b624-c7d4418298d0\"},{\"content\":{\"connectorIds\":[\"LConn1\"],\"side\":\"TOP\"},\"type\":\"ConnectorPlacement.EquallySpacedRectSide\",\"uuid\":\"a3401fa4-31f5-4c91-8a09-9f2730c54d6f\"},{\"content\":{\"connectorIds\":[\"RConn1\"],\"side\":\"BOTTOM\"},\"type\":\"ConnectorPlacement.EquallySpacedRectSide\",\"uuid\":\"ec3e6ca2-4822-4b63-8ee1-1049d14efe1d\"}]},\"type\":\"ConnectorPlacement.EquallySpacedConnector\",\"uuid\":\"06f44f8b-bef4-44e1-af36-23832e4d595a\"}],\"packageUris\":[\"http://schema.mathworks.com/mf0/Connector/R2020b\"],\"version\":\"1.0\"}"
  K : PMIOPort  Side=Right
  A : PMIOPort  Port=2  Side=Left
  connections:
  D12/LConn1 -- K/RConn1
  A/RConn1 -- D12/RConn1

== system six_pulse_dstack_based_rectifier/six_pulse rectifier/BR2/ssc_diode_rr_bridge/D6/D13 ==
  D13 : Subsystem
      settings: PortSchema="{\"entries\":[{\"content\":{\"sides\":[{\"content\":{},\"type\":\"ConnectorPlacement.EquallySpacedRectSide\",\"uuid\":\"7269b907-ab9b-4481-ac18-a8dd984c3818\"},{\"content\":{\"side\":\"RIGHT\"},\"type\":\"ConnectorPlacement.EquallySpacedRectSide\",\"uuid\":\"8dceca02-62a3-4342-b624-c7d4418298d0\"},{\"content\":{\"connectorIds\":[\"LConn1\"],\"side\":\"TOP\"},\"type\":\"ConnectorPlacement.EquallySpacedRectSide\",\"uuid\":\"a3401fa4-31f5-4c91-8a09-9f2730c54d6f\"},{\"content\":{\"connectorIds\":[\"RConn1\"],\"side\":\"BOTTOM\"},\"type\":\"ConnectorPlacement.EquallySpacedRectSide\",\"uuid\":\"ec3e6ca2-4822-4b63-8ee1-1049d14efe1d\"}]},\"type\":\"ConnectorPlacement.EquallySpacedConnector\",\"uuid\":\"06f44f8b-bef4-44e1-af36-23832e4d595a\"}],\"packageUris\":[\"http://schema.mathworks.com/mf0/Connector/R2020b\"],\"version\":\"1.0\"}"
  K : PMIOPort  Side=Right
  A : PMIOPort  Port=2  Side=Left
  connections:
  A/RConn1 -- D13/RConn1
  D13/LConn1 -- K/RConn1

== system six_pulse_dstack_based_rectifier/six_pulse rectifier/BR2/ssc_diode_rr_bridge/D6/D14 ==
  D14 : Subsystem
      settings: PortSchema="{\"entries\":[{\"content\":{\"sides\":[{\"content\":{},\"type\":\"ConnectorPlacement.EquallySpacedRectSide\",\"uuid\":\"7269b907-ab9b-4481-ac18-a8dd984c3818\"},{\"content\":{\"side\":\"RIGHT\"},\"type\":\"ConnectorPlacement.EquallySpacedRectSide\",\"uuid\":\"8dceca02-62a3-4342-b624-c7d4418298d0\"},{\"content\":{\"connectorIds\":[\"LConn1\"],\"side\":\"TOP\"},\"type\":\"ConnectorPlacement.EquallySpacedRectSide\",\"uuid\":\"a3401fa4-31f5-4c91-8a09-9f2730c54d6f\"},{\"content\":{\"connectorIds\":[\"RConn1\"],\"side\":\"BOTTOM\"},\"type\":\"ConnectorPlacement.EquallySpacedRectSide\",\"uuid\":\"ec3e6ca2-4822-4b63-8ee1-1049d14efe1d\"}]},\"type\":\"ConnectorPlacement.EquallySpacedConnector\",\"uuid\":\"06f44f8b-bef4-44e1-af36-23832e4d595a\"}],\"packageUris\":[\"http://schema.mathworks.com/mf0/Connector/R2020b\"],\"version\":\"1.0\"}"
  K : PMIOPort  Side=Right
  A : PMIOPort  Port=2  Side=Left
  connections:
  D14/LConn1 -- K/RConn1
  A/RConn1 -- D14/RConn1

== system six_pulse_dstack_based_rectifier/six_pulse rectifier/BR2/ssc_diode_rr_bridge/D6/D15 ==
  D15 : Subsystem
      settings: PortSchema="{\"entries\":[{\"content\":{\"sides\":[{\"content\":{},\"type\":\"ConnectorPlacement.EquallySpacedRectSide\",\"uuid\":\"7269b907-ab9b-4481-ac18-a8dd984c3818\"},{\"content\":{\"side\":\"RIGHT\"},\"type\":\"ConnectorPlacement.EquallySpacedRectSide\",\"uuid\":\"8dceca02-62a3-4342-b624-c7d4418298d0\"},{\"content\":{\"connectorIds\":[\"LConn1\"],\"side\":\"TOP\"},\"type\":\"ConnectorPlacement.EquallySpacedRectSide\",\"uuid\":\"a3401fa4-31f5-4c91-8a09-9f2730c54d6f\"},{\"content\":{\"connectorIds\":[\"RConn1\"],\"side\":\"BOTTOM\"},\"type\":\"ConnectorPlacement.EquallySpacedRectSide\",\"uuid\":\"ec3e6ca2-4822-4b63-8ee1-1049d14efe1d\"}]},\"type\":\"ConnectorPlacement.EquallySpacedConnector\",\"uuid\":\"06f44f8b-bef4-44e1-af36-23832e4d595a\"}],\"packageUris\":[\"http://schema.mathworks.com/mf0/Connector/R2020b\"],\"version\":\"1.0\"}"
  K : PMIOPort  Side=Right
  A : PMIOPort  Port=2  Side=Left
  connections:
  A/RConn1 -- D15/RConn1
  D15/LConn1 -- K/RConn1

== system six_pulse_dstack_based_rectifier/six_pulse rectifier/BR2/ssc_diode_rr_bridge/D6/D16 ==
  D16 : Subsystem
      settings: PortSchema="{\"entries\":[{\"content\":{\"sides\":[{\"content\":{},\"type\":\"ConnectorPlacement.EquallySpacedRectSide\",\"uuid\":\"7269b907-ab9b-4481-ac18-a8dd984c3818\"},{\"content\":{\"side\":\"RIGHT\"},\"type\":\"ConnectorPlacement.EquallySpacedRectSide\",\"uuid\":\"8dceca02-62a3-4342-b624-c7d4418298d0\"},{\"content\":{\"connectorIds\":[\"LConn1\"],\"side\":\"TOP\"},\"type\":\"ConnectorPlacement.EquallySpacedRectSide\",\"uuid\":\"a3401fa4-31f5-4c91-8a09-9f2730c54d6f\"},{\"content\":{\"connectorIds\":[\"RConn1\"],\"side\":\"BOTTOM\"},\"type\":\"ConnectorPlacement.EquallySpacedRectSide\",\"uuid\":\"ec3e6ca2-4822-4b63-8ee1-1049d14efe1d\"}]},\"type\":\"ConnectorPlacement.EquallySpacedConnector\",\"uuid\":\"06f44f8b-bef4-44e1-af36-23832e4d595a\"}],\"packageUris\":[\"http://schema.mathworks.com/mf0/Connector/R2020b\"],\"version\":\"1.0\"}"
  K : PMIOPort  Side=Right
  A : PMIOPort  Port=2  Side=Left
  connections:
  D16/LConn1 -- K/RConn1
  A/RConn1 -- D16/RConn1

== system six_pulse_dstack_based_rectifier/six_pulse rectifier/BR2/ssc_diode_rr_bridge/D1/D11/D11 ==
  Capacitor : fl_lib/Electrical/Electrical Elements/Capacitor  c=Csnubber_m F  r=Rsnubber_m Ohm  g=0 1/Ohm  i_specify=off  i_priority=None  i=0 A  i_nominal_specify=off  i_nominal_value=1  i_nominal_unit=A  v_specify=off  v_priority=None  v=0 V  v_nominal_specify=off  v_nominal_value=1  v_nominal_unit=V  vc_specify=off  vc_priority=High  vc=0 V  vc_nominal_specify=off  vc_nominal_value=1  vc_nominal_unit=V
  Current Sensor : fl_lib/Electrical/Electrical Sensors/Current Sensor
  Current Sensor1 : fl_lib/Electrical/Electrical Sensors/Current Sensor
  PS-Simulink Converter : nesl_utility/PS-Simulink Converter  PhysicalDomain=network_engine_domain  SubClassName=ps_output  LeftPortType=input  RightPortType=output  PseudoPeriodic=off  Frequencies=[]  VectorFormat=1-D array  Unit=A  AffineConversion=off
  PS-Simulink Converter1 : nesl_utility/PS-Simulink Converter  PhysicalDomain=network_engine_domain  SubClassName=ps_output  LeftPortType=input  RightPortType=output  PseudoPeriodic=off  Frequencies=[]  VectorFormat=1-D array  Unit=V  AffineConversion=off
  PS-Simulink Converter2 : nesl_utility/PS-Simulink Converter  PhysicalDomain=network_engine_domain  SubClassName=ps_output  LeftPortType=input  RightPortType=output  PseudoPeriodic=off  Frequencies=[]  VectorFormat=1-D array  Unit=A  AffineConversion=off
  RR Diode (Lauritzen-Ma) : diode_rr_lib/RR Diode (Lauritzen-Ma)  Is=5e-9 A  N=2  Vt=26e-3 V  tau=350e-9 s  TM=60e-9 s  Rs=0.5e-3 Ohm  Cj0=10e-9 F  Vjp=0.7 V  mg=0.5  FC=0.5  dsm=10e-3 V  i_specify=off  i_priority=None  i=0 A  i_nominal_specify=off  i_nominal_value=1  i_nominal_unit=A  v_specify=off  v_priority=None  v=0 V  v_nominal_specify=off  v_nominal_value=1  v_nominal_unit=V  vj_specify=off  vj_priority=None  vj=0 V  vj_nominal_specify=off  vj_nominal_value=1  vj_nominal_unit=V  qE_specify=off  qE_priority=None  qE=0 C  qE_nominal_specify=off  qE_nominal_value=1e-4  qE_nominal_unit=C  qM_specify=off  qM_priority=High  qM=0 C  qM_nominal_specify=off  qM_nominal_value=1e-4  qM_nominal_unit=C  qj_specify=off  qj_priority=None  qj=0 C  qj_nominal_specify=off  qj_nominal_value=1e-5  qj_nominal_unit=C
  Voltage Sensor : fl_lib/Electrical/Electrical Sensors/Voltage Sensor
  K : PMIOPort  Side=Left
  A : PMIOPort  Port=2  Side=Right
  tag scope: D11_Id=scoped, D11_Ud=scoped, RC11_Id=scoped
  wires:
  PS-Simulink Converter/1 -> [D11_Id]
  PS-Simulink Converter2/1 -> [RC11_Id]
  PS-Simulink Converter1/1 -> [D11_Ud]
  connections:
  Voltage Sensor/RConn2 -- K/RConn1 -- Capacitor/LConn1 -- RR Diode (Lauritzen-Ma)/RConn1
  PS-Simulink Converter1/LConn1 -- Voltage Sensor/RConn1
  PS-Simulink Converter/LConn1 -- Current Sensor/RConn1
  Current Sensor1/RConn2 -- Capacitor/RConn1
  Voltage Sensor/LConn1 -- Current Sensor1/LConn1 -- Current Sensor/RConn2 -- RR Diode (Lauritzen-Ma)/LConn1
  PS-Simulink Converter2/LConn1 -- Current Sensor1/RConn1
  A/RConn1 -- Current Sensor/LConn1

== system six_pulse_dstack_based_rectifier/six_pulse rectifier/BR2/ssc_diode_rr_bridge/D1/D12/D12 ==
  Capacitor : fl_lib/Electrical/Electrical Elements/Capacitor  c=Csnubber_m F  r=Rsnubber_m Ohm  g=0 1/Ohm  i_specify=off  i_priority=None  i=0 A  i_nominal_specify=off  i_nominal_value=1  i_nominal_unit=A  v_specify=off  v_priority=None  v=0 V  v_nominal_specify=off  v_nominal_value=1  v_nominal_unit=V  vc_specify=off  vc_priority=High  vc=0 V  vc_nominal_specify=off  vc_nominal_value=1  vc_nominal_unit=V
  Current Sensor : fl_lib/Electrical/Electrical Sensors/Current Sensor
  Current Sensor1 : fl_lib/Electrical/Electrical Sensors/Current Sensor
  PS-Simulink Converter : nesl_utility/PS-Simulink Converter  PhysicalDomain=network_engine_domain  SubClassName=ps_output  LeftPortType=input  RightPortType=output  PseudoPeriodic=off  Frequencies=[]  VectorFormat=1-D array  Unit=A  AffineConversion=off
  PS-Simulink Converter1 : nesl_utility/PS-Simulink Converter  PhysicalDomain=network_engine_domain  SubClassName=ps_output  LeftPortType=input  RightPortType=output  PseudoPeriodic=off  Frequencies=[]  VectorFormat=1-D array  Unit=V  AffineConversion=off
  PS-Simulink Converter2 : nesl_utility/PS-Simulink Converter  PhysicalDomain=network_engine_domain  SubClassName=ps_output  LeftPortType=input  RightPortType=output  PseudoPeriodic=off  Frequencies=[]  VectorFormat=1-D array  Unit=A  AffineConversion=off
  RR Diode (Lauritzen-Ma) : diode_rr_lib/RR Diode (Lauritzen-Ma)  Is=5e-9 A  N=2  Vt=26e-3 V  tau=350e-9 s  TM=60e-9 s  Rs=0.5e-3 Ohm  Cj0=10e-9 F  Vjp=0.7 V  mg=0.5  FC=0.5  dsm=10e-3 V  i_specify=off  i_priority=None  i=0 A  i_nominal_specify=off  i_nominal_value=1  i_nominal_unit=A  v_specify=off  v_priority=None  v=0 V  v_nominal_specify=off  v_nominal_value=1  v_nominal_unit=V  vj_specify=off  vj_priority=None  vj=0 V  vj_nominal_specify=off  vj_nominal_value=1  vj_nominal_unit=V  qE_specify=off  qE_priority=None  qE=0 C  qE_nominal_specify=off  qE_nominal_value=1e-4  qE_nominal_unit=C  qM_specify=off  qM_priority=High  qM=0 C  qM_nominal_specify=off  qM_nominal_value=1e-4  qM_nominal_unit=C  qj_specify=off  qj_priority=None  qj=0 C  qj_nominal_specify=off  qj_nominal_value=1e-5  qj_nominal_unit=C
  Voltage Sensor : fl_lib/Electrical/Electrical Sensors/Voltage Sensor
  K : PMIOPort  Side=Left
  A : PMIOPort  Port=2  Side=Right
  tag scope: D12_Id=scoped, D12_Ud=scoped, RC12_Id=scoped
  wires:
  PS-Simulink Converter1/1 -> [D12_Ud]
  PS-Simulink Converter2/1 -> [RC12_Id]
  PS-Simulink Converter/1 -> [D12_Id]
  connections:
  A/RConn1 -- Current Sensor/LConn1
  PS-Simulink Converter2/LConn1 -- Current Sensor1/RConn1
  RR Diode (Lauritzen-Ma)/LConn1 -- Current Sensor/RConn2 -- Current Sensor1/LConn1 -- Voltage Sensor/LConn1
  Current Sensor1/RConn2 -- Capacitor/RConn1
  PS-Simulink Converter/LConn1 -- Current Sensor/RConn1
  PS-Simulink Converter1/LConn1 -- Voltage Sensor/RConn1
  RR Diode (Lauritzen-Ma)/RConn1 -- Capacitor/LConn1 -- Voltage Sensor/RConn2 -- K/RConn1
